simulink model "impmodel"  (R2023a)
settings: Solver=FixedStepDiscrete  StartTime=0.0  StopTime=8  RelTol=1e-3  EnableMultiTasking=on
values from neighbouring files (symbols this model uses):
  availableSpeedModes = 3    [params_f2838.mat]
  inverter_DRV8300 =     [params_f2838.mat]
  PI_params =     [params_f2838.mat]
  pmsm_ECI6360 =     [params_f2838.mat]
  PU_System =     [params_f2838.mat]
  target_f2838 =     [params_f2838.mat]
  Ts = 5e-05    [params_f2838.mat]
  Ts_motor = 2.5e-05    [params_f2838.mat]
  Ts_simulink = 2.5e-05    [params_f2838.mat]
  Ts_speed = 0.0005    [params_f2838.mat]
undefined symbols (not defined in the file or in its folder): Down, GPTRIP1SEL, TZ1, Up
libraries: simulink x35, c2802xlib x11, idelinklib_common x8, procinterlib x8, mcbcontrolslib x8, c280xlib x7, mcbpositiondecoderlib x7, slpidlib x5, svdschedulerlib x4, c2838xlib x2, autolibpmsminterior x1, mcbplantlib x1
(part 3 of 4)

== system impmodel/Torque Controller/Output/CodeGeneration ==
  In1 : Inport
  Demux : Demux  Outputs=6
  Gain : Gain  Gain=target_f2838.PWM_Counter_Period  OutDataTypeStr=fixdt(1,32,17)
  ePWM1 : c2802xlib/ePWM  PwmType=C2000_Type4_F2838x  useModule=ePWM6  ePWMxLINKTBPRD=Not Linked  periodUnits=Clock cycles  timerSource=Specify via dialog  timerPeriod_clk=target_f2838.PWM_Counter_Period  timerPeriod_sec=0.0001  tbshadow=Counter equals to zero  countingMode=Up-Down  phaseActiveEnable=Disable  phaseDirection=Count down after sync  phaseActive=0  synchronizationEnable=off  dcaevt1Sync=off  dcbevt1Sync=off  synchronizationOption=Disable  dcbevt1SyncOut=off  dcaevt1SyncOut=off  cmpdSyncOut=off  cmpcSyncOut=off  cmpbSyncOut=off  zeroSyncOut=on  swfSyncOut=off  perSynchronizationOption=Counter equals to period (CTR=PRD)  clockPrescale=1  HSclockPrescale=1  enswap=off  ePWMxAStatus=on  ePWMxAactionLogic1=Do nothing  ePWMxAactionLogic2=Do nothing  ePWMxAactionLogic3=Clear  ePWMxAactionLogic4=Set  ePWMxAactionLogic5=Do nothing  ePWMxAactionLogic6=Do nothing  ePWMxACSFenable=off  ePWMxACSFvalue=Forcing disable  ePWMxASFreload=Zero  ePWMxBStatus=on  ePWMxBactionLogic1=Do nothing  ePWMxBactionLogic2=Do nothing  ePWMxBactionLogic3=Do nothing  ePWMxBactionLogic4=Do nothing  ePWMxBactionLogic5=Clear  ePWMxBactionLogic6=Set  ePWMxBCSFenable=off  ePWMxBCSFvalue=Forcing disable  ePWMxBSFreload=Zero  ePWNxBOutWay=off  ePWMxLINKCMPA=Not Linked  CMPAUnits=Clock cycles  CMPASource=Input port  CMPAValue_per=50  CMPAValue_clk=floor(target_f2838.PWM_Counter_Period/2)  enCMPAshadow=Counter equals to zero (CTR=Zero)  ePWMxLINKCMPB=Not Linked  CMPBUnits=Clock cycles  CMPBSource=Input port  CMPBValue_per=50  CMPBValue_clk=floor(target_f2838.PWM_Counter_Period/2)  enCMPBshadow=Counter equals to zero (CTR=Zero)  ePWMxLINKCMPC=Not Linked  CMPCUnits=Clock cycles  CMPCSource=Specify via dialog  CMPCValue_per=50  CMPCValue_clk=32000  enCMPCshadow=Counter equals to zero (CTR=Zero)  ePWMxLINKCMPD=Not Linked  CMPDUnits=Clock cycles  CMPDSource=Specify via dialog  CMPDValue_per=50  CMPDValue_clk=32000  enCMPDshadow=Counter equals to zero (CTR=Zero)  enableDBePWMxA=off  enableDBePWMxB=off  enhalfcycle=off  DBpolarity=Active high complementary (AHC)  DBedgeDelay=Positive  DBSource_ePWMxA=ePWMxA  DBSource_ePWMxB=ePWMxA  DBPeriodUnits=Clock cycles  DBperiodSource=Specify via dialog  REDperiod=15  FEDperiod=15  REDperiod_sec=0  FEDperiod_sec=0  LoadModeDBRED=Immediate without using shadow  LoadModeDBFED=Immediate without using shadow  adcstartModuleA=on  adcrequestEventA=First event  adcstartEventA=Digital Compare Module A Event 1 start of conversion (DCAEVT1.soc)  adcstartEventA_type2=Counter equals to period (CTR=PRD)  adcstartModuleB=off  adcrequestEventB=First event  adcstartEventB=Counter equals to zero (CTR=Zero)  adcstartEventB_type2=Counter equals to zero (CTR=Zero)  intEn=off  intPrd=First event  intSel=Counter equals to zero (CTR=Zero)  intSel_type2=Counter equals to zero (CTR=Zero)  hrpe=off  enHRPWM=off  HRPWM_LoadMode=Counter equals to period (CTR=PRD)  HRPWM_CTLMode=Duty or Period control mode  HRPWM_EDGMode=Both edge  hrpeb=off  enHRPWMB=off  HRPWM_LoadModeB=Counter equals to zero (CTR=ZERO)  HRPWM_CTLModeB=Duty or Period control mode  HRPWM_EDGModeB=Both edge  enHRDBRED=off  enHRDBFED=off  enSFO=on  enautoconv=on  chopperEnable=off  chopperFrequency=1  chopperFirstwidth=1  chopperDuty=12.5%  tripZonesource=Specify via dialog  tzselOSHT1=off  tzselOSHT2=off  tzselOSHT3=off  tzselOSHDCAEV1=off  tzselOSHDCBEV1=off  tzselCBC1=off  tzselCBC2=off  tzselCBC3=off  tzselCBCDCAEV2=off  tzselCBCDCBEV2=off  tzselOSHT4=off  tzselOSHT5=off  tzselOSHT6=off  tzselCBC4=off  tzselCBC5=off  tzselCBC6=off  enTzOstIntr=off  enTzCbcIntr=off  enTzDCAEVT1Intr=off  enTzDCAEVT2Intr=off  enTzDCBEVT1Intr=off  enTzDCBEVT2Intr=off  ePWMxAforced=No action  ePWMxBforced=No action  DCAEVT1forced=No action  DCBEVT1forced=No action  DCAEVT2forced=No action  DCBEVT2forced=No action  dcah=Trip Zone 1 input (TZ1)  dcal=Trip Zone 2 input (TZ2)  dcbh=Trip Zone 1 input (TZ1)  dcbl=Trip Zone 2 input (TZ2)  dcah_type2=GPTRIP1SEL/(TZ1)  dcal_type2=GPTRIP1SEL/(TZ1)  dcbh_type2=GPTRIP1SEL/(TZ1)  dcbl_type2=GPTRIP1SEL/(TZ1)  gendcaevt1=Event disabled  gendcaevt2=Event disabled  gendcbevt1=Event disabled  gendcbevt2=Event disabled  dcaevt1src=DCAEVT1 with sync  dcaevt2src=DCAEVT2 with sync  dcbevt1src=DCBEVT1 with sync  dcbevt2src=DCBEVT2 with sync  pulsesel=Counter equals to zero (CTR=Zero)  blankinv=off  blankoffset=0  blankwidth=0  evsrcsel=Filtered version of DCAEVT1 (DCAEVT1FILT)  encape=off
      settings: LibrarySourceBlock=c2838xlib/ePWM
  ePWM2 : c2802xlib/ePWM  PwmType=C2000_Type4_F2838x  useModule=ePWM7  ePWMxLINKTBPRD=Not Linked  periodUnits=Clock cycles  timerSource=Specify via dialog  timerPeriod_clk=target_f2838.PWM_Counter_Period  timerPeriod_sec=0.0001  tbshadow=Counter equals to zero  countingMode=Up-Down  phaseActiveEnable=Set counter to phase value specified via dialog  phaseDirection=Count up after sync  phaseActive=0  synchronizationEnable=off  dcaevt1Sync=off  dcbevt1Sync=off  synchronizationOption=Disable  dcbevt1SyncOut=off  dcaevt1SyncOut=off  cmpdSyncOut=off  cmpcSyncOut=off  cmpbSyncOut=off  zeroSyncOut=off  swfSyncOut=on  perSynchronizationOption=Counter equals to period (CTR=PRD)  clockPrescale=1  HSclockPrescale=1  enswap=off  ePWMxAStatus=on  ePWMxAactionLogic1=Do nothing  ePWMxAactionLogic2=Do nothing  ePWMxAactionLogic3=Clear  ePWMxAactionLogic4=Set  ePWMxAactionLogic5=Do nothing  ePWMxAactionLogic6=Do nothing  ePWMxACSFenable=off  ePWMxACSFvalue=Forcing disable  ePWMxASFreload=Zero  ePWMxBStatus=on  ePWMxBactionLogic1=Do nothing  ePWMxBactionLogic2=Do nothing  ePWMxBactionLogic3=Do nothing  ePWMxBactionLogic4=Do nothing  ePWMxBactionLogic5=Clear  ePWMxBactionLogic6=Set  ePWMxBCSFenable=off  ePWMxBCSFvalue=Forcing disable  ePWMxBSFreload=Zero  ePWNxBOutWay=off  ePWMxLINKCMPA=Not Linked  CMPAUnits=Clock cycles  CMPASource=Input port  CMPAValue_per=50  CMPAValue_clk=floor(target_f2838.PWM_Counter_Period/2)  enCMPAshadow=Counter equals to zero (CTR=Zero)  ePWMxLINKCMPB=Not Linked  CMPBUnits=Clock cycles  CMPBSource=Input port  CMPBValue_per=50  CMPBValue_clk=floor(target_f2838.PWM_Counter_Period/2)  enCMPBshadow=Counter equals to zero (CTR=Zero)  ePWMxLINKCMPC=Not Linked  CMPCUnits=Clock cycles  CMPCSource=Specify via dialog  CMPCValue_per=50  CMPCValue_clk=32000  enCMPCshadow=Counter equals to zero (CTR=Zero)  ePWMxLINKCMPD=Not Linked  CMPDUnits=Clock cycles  CMPDSource=Specify via dialog  CMPDValue_per=50  CMPDValue_clk=32000  enCMPDshadow=Counter equals to zero (CTR=Zero)  enableDBePWMxA=off  enableDBePWMxB=off  enhalfcycle=off  DBpolarity=Active high complementary (AHC)  DBedgeDelay=Positive  DBSource_ePWMxA=ePWMxA  DBSource_ePWMxB=ePWMxA  DBPeriodUnits=Clock cycles  DBperiodSource=Specify via dialog  REDperiod=15  FEDperiod=15  REDperiod_sec=0  FEDperiod_sec=0  LoadModeDBRED=Immediate without using shadow  LoadModeDBFED=Immediate without using shadow  adcstartModuleA=off  adcrequestEventA=First event  adcstartEventA=Digital Compare Module A Event 1 start of conversion (DCAEVT1.soc)  adcstartEventA_type2=Counter equals to zero (CTR=Zero)  adcstartModuleB=off  adcrequestEventB=First event  adcstartEventB=Counter equals to zero (CTR=Zero)  adcstartEventB_type2=Counter equals to zero (CTR=Zero)  intEn=off  intPrd=First event  intSel=Counter equals to zero (CTR=Zero)  intSel_type2=Counter equals to zero (CTR=Zero)  hrpe=off  enHRPWM=off  HRPWM_LoadMode=Counter equals to period (CTR=PRD)  HRPWM_CTLMode=Duty or Period control mode  HRPWM_EDGMode=Both edge  hrpeb=off  enHRPWMB=off  HRPWM_LoadModeB=Counter equals to zero (CTR=ZERO)  HRPWM_CTLModeB=Duty or Period control mode  HRPWM_EDGModeB=Both edge  enHRDBRED=off  enHRDBFED=off  enSFO=on  enautoconv=on  chopperEnable=off  chopperFrequency=1  chopperFirstwidth=1  chopperDuty=12.5%  tripZonesource=Specify via dialog  tzselOSHT1=off  tzselOSHT2=off  tzselOSHT3=off  tzselOSHDCAEV1=off  tzselOSHDCBEV1=off  tzselCBC1=off  tzselCBC2=off  tzselCBC3=off  tzselCBCDCAEV2=off  tzselCBCDCBEV2=off  tzselOSHT4=off  tzselOSHT5=off  tzselOSHT6=off  tzselCBC4=off  tzselCBC5=off  tzselCBC6=off  enTzOstIntr=off  enTzCbcIntr=off  enTzDCAEVT1Intr=off  enTzDCAEVT2Intr=off  enTzDCBEVT1Intr=off  enTzDCBEVT2Intr=off  ePWMxAforced=No action  ePWMxBforced=No action  DCAEVT1forced=No action  DCBEVT1forced=No action  DCAEVT2forced=No action  DCBEVT2forced=No action  dcah=Trip Zone 1 input (TZ1)  dcal=Trip Zone 2 input (TZ2)  dcbh=Trip Zone 1 input (TZ1)  dcbl=Trip Zone 2 input (TZ2)  dcah_type2=GPTRIP1SEL/(TZ1)  dcal_type2=GPTRIP1SEL/(TZ1)  dcbh_type2=GPTRIP1SEL/(TZ1)  dcbl_type2=GPTRIP1SEL/(TZ1)  gendcaevt1=Event disabled  gendcaevt2=Event disabled  gendcbevt1=Event disabled  gendcbevt2=Event disabled  dcaevt1src=DCAEVT1 with sync  dcaevt2src=DCAEVT2 with sync  dcbevt1src=DCBEVT1 with sync  dcbevt2src=DCBEVT2 with sync  pulsesel=Counter equals to zero (CTR=Zero)  blankinv=off  blankoffset=0  blankwidth=0  evsrcsel=Filtered version of DCAEVT1 (DCAEVT1FILT)  encape=off
      settings: LibrarySourceBlock=c2838xlib/ePWM
  ePWM3 : c2802xlib/ePWM  PwmType=C2000_Type4_F2838x  useModule=ePWM8  ePWMxLINKTBPRD=Not Linked  periodUnits=Clock cycles  timerSource=Specify via dialog  timerPeriod_clk=target_f2838.PWM_Counter_Period  timerPeriod_sec=0.0001  tbshadow=Counter equals to zero  countingMode=Up-Down  phaseActiveEnable=Set counter to phase value specified via dialog  phaseDirection=Count up after sync  phaseActive=0  synchronizationEnable=off  dcaevt1Sync=off  dcbevt1Sync=off  synchronizationOption=Disable  dcbevt1SyncOut=off  dcaevt1SyncOut=off  cmpdSyncOut=off  cmpcSyncOut=off  cmpbSyncOut=off  zeroSyncOut=off  swfSyncOut=on  perSynchronizationOption=Counter equals to period (CTR=PRD)  clockPrescale=1  HSclockPrescale=1  enswap=off  ePWMxAStatus=on  ePWMxAactionLogic1=Do nothing  ePWMxAactionLogic2=Do nothing  ePWMxAactionLogic3=Clear  ePWMxAactionLogic4=Set  ePWMxAactionLogic5=Do nothing  ePWMxAactionLogic6=Do nothing  ePWMxACSFenable=off  ePWMxACSFvalue=Forcing disable  ePWMxASFreload=Zero  ePWMxBStatus=on  ePWMxBactionLogic1=Do nothing  ePWMxBactionLogic2=Do nothing  ePWMxBactionLogic3=Do nothing  ePWMxBactionLogic4=Do nothing  ePWMxBactionLogic5=Clear  ePWMxBactionLogic6=Set  ePWMxBCSFenable=off  ePWMxBCSFvalue=Forcing disable  ePWMxBSFreload=Zero  ePWNxBOutWay=off  ePWMxLINKCMPA=Not Linked  CMPAUnits=Clock cycles  CMPASource=Input port  CMPAValue_per=50  CMPAValue_clk=floor(target_f2838.PWM_Counter_Period/2)  enCMPAshadow=Counter equals to zero (CTR=Zero)  ePWMxLINKCMPB=Not Linked  CMPBUnits=Clock cycles  CMPBSource=Input port  CMPBValue_per=50  CMPBValue_clk=floor(target_f2838.PWM_Counter_Period/2)  enCMPBshadow=Counter equals to zero (CTR=Zero)  ePWMxLINKCMPC=Not Linked  CMPCUnits=Clock cycles  CMPCSource=Specify via dialog  CMPCValue_per=50  CMPCValue_clk=32000  enCMPCshadow=Counter equals to zero (CTR=Zero)  ePWMxLINKCMPD=Not Linked  CMPDUnits=Clock cycles  CMPDSource=Specify via dialog  CMPDValue_per=50  CMPDValue_clk=32000  enCMPDshadow=Counter equals to zero (CTR=Zero)  enableDBePWMxA=off  enableDBePWMxB=off  enhalfcycle=off  DBpolarity=Active high complementary (AHC)  DBedgeDelay=Positive  DBSource_ePWMxA=ePWMxA  DBSource_ePWMxB=ePWMxA  DBPeriodUnits=Clock cycles  DBperiodSource=Specify via dialog  REDperiod=15  FEDperiod=15  REDperiod_sec=0  FEDperiod_sec=0  LoadModeDBRED=Immediate without using shadow  LoadModeDBFED=Immediate without using shadow  adcstartModuleA=off  adcrequestEventA=First event  adcstartEventA=Digital Compare Module A Event 1 start of conversion (DCAEVT1.soc)  adcstartEventA_type2=Counter equals to zero (CTR=Zero)  adcstartModuleB=off  adcrequestEventB=First event  adcstartEventB=Counter equals to zero (CTR=Zero)  adcstartEventB_type2=Counter equals to zero (CTR=Zero)  intEn=off  intPrd=First event  intSel=Counter equals to zero (CTR=Zero)  intSel_type2=Counter equals to zero (CTR=Zero)  hrpe=off  enHRPWM=off  HRPWM_LoadMode=Counter equals to period (CTR=PRD)  HRPWM_CTLMode=Duty or Period control mode  HRPWM_EDGMode=Both edge  hrpeb=off  enHRPWMB=off  HRPWM_LoadModeB=Counter equals to zero (CTR=ZERO)  HRPWM_CTLModeB=Duty or Period control mode  HRPWM_EDGModeB=Both edge  enHRDBRED=off  enHRDBFED=off  enSFO=on  enautoconv=on  chopperEnable=off  chopperFrequency=1  chopperFirstwidth=1  chopperDuty=12.5%  tripZonesource=Specify via dialog  tzselOSHT1=off  tzselOSHT2=off  tzselOSHT3=off  tzselOSHDCAEV1=off  tzselOSHDCBEV1=off  tzselCBC1=off  tzselCBC2=off  tzselCBC3=off  tzselCBCDCAEV2=off  tzselCBCDCBEV2=off  tzselOSHT4=off  tzselOSHT5=off  tzselOSHT6=off  tzselCBC4=off  tzselCBC5=off  tzselCBC6=off  enTzOstIntr=off  enTzCbcIntr=off  enTzDCAEVT1Intr=off  enTzDCAEVT2Intr=off  enTzDCBEVT1Intr=off  enTzDCBEVT2Intr=off  ePWMxAforced=No action  ePWMxBforced=No action  DCAEVT1forced=No action  DCBEVT1forced=No action  DCAEVT2forced=No action  DCBEVT2forced=No action  dcah=Trip Zone 1 input (TZ1)  dcal=Trip Zone 2 input (TZ2)  dcbh=Trip Zone 1 input (TZ1)  dcbl=Trip Zone 2 input (TZ2)  dcah_type2=GPTRIP1SEL/(TZ1)  dcal_type2=GPTRIP1SEL/(TZ1)  dcbh_type2=GPTRIP1SEL/(TZ1)  dcbl_type2=GPTRIP1SEL/(TZ1)  gendcaevt1=Event disabled  gendcaevt2=Event disabled  gendcbevt1=Event disabled  gendcbevt2=Event disabled  dcaevt1src=DCAEVT1 with sync  dcaevt2src=DCAEVT2 with sync  dcbevt1src=DCBEVT1 with sync  dcbevt2src=DCBEVT2 with sync  pulsesel=Counter equals to zero (CTR=Zero)  blankinv=off  blankoffset=0  blankwidth=0  evsrcsel=Filtered version of DCAEVT1 (DCAEVT1FILT)  encape=off
      settings: LibrarySourceBlock=c2838xlib/ePWM
  wires:
  In1/1 -> Gain/1
  Demux/1 -> ePWM1/1
  Demux/6 -> ePWM3/2
  Demux/2 -> ePWM1/2
  Demux/5 -> ePWM3/1
  Demux/4 -> ePWM2/2
  Demux/3 -> ePWM2/1
  Gain/1 -> Demux/1

== system impmodel/Torque Controller/Output/Simulation ==
  Input : Inport
  Demux : Demux  Outputs=6
  Mux : Mux  Inputs=3
  Terminator : Terminator
  Terminator1 : Terminator
  Terminator2 : Terminator
  Output : Outport
  wires:
  Demux/5 -> Mux/3
  Demux/4 -> Terminator1/1
  Demux/1 -> Mux/1
  Demux/6 -> Terminator/1
  Demux/2 -> Terminator2/1
  Demux/3 -> Mux/2
  Input/1 -> Demux/1
  Mux/1 -> Output/1

== system impmodel/Torque Controller/Scaling DutyCycles/CodeGen ==
  In1 : Inport
  Constant : Constant  Value=0.5  OutDataTypeStr=fixdt(1,32,17)  SampleTime=-1
  Gain : Gain  Gain=-0.5  RndMeth=Simplest  OutDataTypeStr=Inherit: Same as input
  Sum : Sum  Inputs=|++
  Out1 : Outport
  wires:
  In1/1 -> Gain/1
  Sum/1 -> Out1/1
  Constant/1 -> Sum/2
  Gain/1 -> Sum/1

== system impmodel/Torque Controller/Scaling DutyCycles/Sim ==
  In1 : Inport
  Constant : Constant  Value=0.5  OutDataTypeStr=fixdt(1,32,17)  SampleTime=-1
  Gain : Gain  Gain=-0.5  RndMeth=Simplest  OutDataTypeStr=Inherit: Same as input
  Sum : Sum  Inputs=|++
  Out1 : Outport
  wires:
  In1/1 -> Gain/1
  Sum/1 -> Out1/1
  Constant/1 -> Sum/2
  Gain/1 -> Sum/1

== system impmodel/Torque Controller/TCP_Position/Data_Type_Fixed_Point ==
  In1 : Inport
  Data Type Conversion : DataTypeConversion  OutDataTypeStr=fixdt(1,32,17)  RndMeth=Simplest  SaturateOnIntegerOverflow=off
  Data Type Conversion3 : DataTypeConversion  OutDataTypeStr=uint32  ConvertRealWorld=Stored Integer (SI)  RndMeth=Simplest  SaturateOnIntegerOverflow=off
  Data_Log : Outport
  wires:
  In1/1 -> Data Type Conversion/1
  Data Type Conversion3/1 -> Data_Log/1
  Data Type Conversion/1 -> Data Type Conversion3/1

== system impmodel/Torque Controller/TCP_Speed/Data_Type_Fixed_Point ==
  In1 : Inport
  Data Type Conversion : DataTypeConversion  OutDataTypeStr=fixdt(1,32,17)  RndMeth=Simplest  SaturateOnIntegerOverflow=off
  Data Type Conversion3 : DataTypeConversion  OutDataTypeStr=uint32  ConvertRealWorld=Stored Integer (SI)  RndMeth=Simplest  SaturateOnIntegerOverflow=off
  Data_Log : Outport
  wires:
  In1/1 -> Data Type Conversion/1
  Data Type Conversion3/1 -> Data_Log/1
  Data Type Conversion/1 -> Data Type Conversion3/1

== system impmodel/ADC Offset Function/Calculate ADC Offset /For Iterator Subsystem/If Action Subsystem ==
  In1 : Inport
  In2 : Inport  Port=2
  Action Port : ActionPort  ActionPortLabel=if(u1 > 8)
  Memory : Memory  InheritSampleTime=on
  Memory1 : Memory  InheritSampleTime=on
  Sum : Sum
  Sum1 : Sum
  Out1 : Outport
  Out2 : Outport  Port=2
  wires:
  In1/1 -> Sum/1
  Sum/1 -> Out1/1, Memory/1
  In2/1 -> Sum1/1
  Memory/1 -> Sum/2
  Sum1/1 -> Out2/1, Memory1/1
  Memory1/1 -> Sum1/2

== system impmodel/Input Controller/SpeedCommand_CodeGen/Check for SpeedRef/If Action Subsystem ==
  Action Port : ActionPort  ActionPortLabel=if(u1 > 4000)
  Constant : Constant  Value=4095  OutDataTypeStr=uint16  SampleTime=-1
  Out1 : Outport
  wires:
  Constant/1 -> Out1/1

== system impmodel/Input Controller/SpeedCommand_CodeGen/Check for SpeedRef/If Action Subsystem1 ==
  In1 : Inport
  Action Port : ActionPort  ActionPortLabel=else
  Out1 : Outport
  wires:
  In1/1 -> Out1/1

== system impmodel/Input Controller/Subsystem/TCP_temp/Data_Type_Fixed_Point ==
  In1 : Inport
  Data Type Conversion : DataTypeConversion  OutDataTypeStr=fixdt(1,32,17)  RndMeth=Simplest  SaturateOnIntegerOverflow=off
  Data Type Conversion3 : DataTypeConversion  OutDataTypeStr=uint32  ConvertRealWorld=Stored Integer (SI)  RndMeth=Simplest  SaturateOnIntegerOverflow=off
  Data_Log : Outport
  wires:
  In1/1 -> Data Type Conversion/1
  Data Type Conversion3/1 -> Data_Log/1
  Data Type Conversion/1 -> Data Type Conversion3/1

== system impmodel/Speed Control/Speed calculator/Subsystem/If Action Subsystem ==
  Action Port : ActionPort
  Constant : Constant  OutDataTypeStr=fixdt(1,32,17)  SampleTime=-1
  Out1 : Outport
  wires:
  Constant/1 -> Out1/1

== system impmodel/Speed Control/Speed calculator/Subsystem/If Action Subsystem1 ==
  In1 : Inport
  Action Port : ActionPort
  Data Type Conversion : DataTypeConversion  OutDataTypeStr=fixdt(1,32,17)  SaturateOnIntegerOverflow=off  RndMeth=Floor
  Out1 : Outport
  wires:
  In1/1 -> Data Type Conversion/1
  Data Type Conversion/1 -> Out1/1

== system impmodel/Torque Controller/FOC/Current_Controllers/PI_Controller_Id ==
  Id_in : Inport
  Data Store Read1 : DataStoreRead  Commented=on  DataStoreName=Enable  IndexOptions=Index vector (dialog)  Indices=1  OutputSizes=1
  Discrete PI Controller with anti-windup & reset : slpidlib/PID Controller  Commented=on  Controller=PI  Form=Parallel  TimeDomain=Discrete-time  UseExternalTs=off  SampleTime=-1  IntegratorMethod=Forward Euler  FilterMethod=Forward Euler  ControllerParametersSource=external  P=1  I=1  UseKiTs=on  D=0  N=100  UseFilter=on  TunerSelectOption=Transfer Function Based (PID Tuner App)  InitialConditionSource=external  InitialConditionForIntegrator=0  InitialConditionForFilter=0  DifferentiatorICPrevScaledInput=0  ExternalReset=level  TrackingMode=off  Kt=1  LimitOutput=on  SatLimitsSource=internal  UpperSaturationLimit=1  LowerSaturationLimit=-1  LinearizeAsGain=on  AntiWindupMode=clamping  Kb=1  LimitIntegrator=off  UpperIntegratorSaturationLimit=inf  LowerIntegratorSaturationLimit=-inf  RndMeth=Simplest  PGainOutDataTypeStr=single  PProdOutDataTypeStr=single  POutMin=[]  POutMax=[]  IGainOutDataTypeStr=single  IProdOutDataTypeStr=single  IOutMin=[]  IOutMax=[]  DOutMin=[]  DOutMax=[]  NOutMin=[]  NOutMax=[]  SumOutDataTypeStr=single  SumOutMin=[]  SumOutMax=[]  SaturationOutDataTypeStr=single  SaturationOutMin=[]  SaturationOutMax=[]  PParamMin=[]  PParamMax=[]  IParamMin=[]  IParamMax=[]  DParamMin=[]  DParamMax=[]  NParamMin=[]  NParamMax=[]  KbParamMin=[]  KbParamMax=[]  KtParamMin=[]  KtParamMax=[]  KbOutMin=[]  KbOutMax=[]  KtOutMin=[]  KtOutMax=[]  IntegratorOutMin=[]  IntegratorOutMax=[]  FilterOutMin=[]  FilterOutMax=[]  SumI1OutMin=[]  SumI1OutMax=[]  SumI2OutMin=[]  SumI2OutMax=[]  SumI3OutMin=[]  SumI3OutMax=[]  SumI4OutMin=[]  SumI4OutMax=[]  SumDOutMin=[]  SumDOutMax=[]  DifferentiatorOutMin=[]  DifferentiatorOutMax=[]  FilterDiffOutCoefMin=[]  FilterDiffOutCoefMax=[]  ReciprocalOutMin=[]  ReciprocalOutMax=[]  SumDenOutMin=[]  SumDenOutMax=[]  SumNumOutMin=[]  SumNumOutMax=[]  DivideOutMin=[]  DivideOutMax=[]  UdiffTsProdOutMin=[]  UdiffTsProdOutMax=[]  NTsProdOutMin=[]  NTsProdOutMax=[]  UintegralTsProdOutMin=[]  UintegralTsProdOutMax=[]  UngainTsProdOutMin=[]  UngainTsProdOutMax=[]  ClampingZeroOutDataTypeStr=Inherit: Inherit via back propagation  ClampingZeroOutMin=[]  ClampingZeroOutMax=[]  FilterDenConstantOutDataTypeStr=Inherit: Inherit via back propagation  FilterDenConstantOutMin=[]  FilterDenConstantOutMax=[]  PCopyOutDataTypeStr=Inherit: Inherit via back propagation  PCopyOutMin=[]  PCopyOutMax=[]  NCopyOutDataTypeStr=Inherit: Inherit via back propagation  NCopyOutMin=[]  NCopyOutMax=[]  IntegratorContinuousStateAttributes=''  IntegratorStateMustResolveToSignalObject=off  IntegratorRTWStateStorageClass=Auto  FilterContinuousStateAttributes=''  FilterStateMustResolveToSignalObject=off  FilterRTWStateStorageClass=Auto  ParallelPVariant=ExternalParameters  IdealPVariant=Disabled  IVariant=ExternalParameters  DVariant=Disabled  IntegratorVariant=Discrete  SatVariant=Enabled  AWVariant=DiscClampingParallel  PCopyVariant=Disabled  TRVariant=Disabled  FdbkBlocksVariant=Forward  IdealPFdbkVariant=Disabled  SatFdbkVariant=Disabled  DerivativeFilterVariant=Disabled  NVariant=Disabled  NCopyVariant=Disabled_SignalSpec  FilterICVariant=Disabled  IntegratorICVariant=ExternalICs  ExternalResetVariant=ExternalReset  TRSumVariant=Passthrough  SumFdbkVariant=Disabled  SumVariant=Sum_PI  TsampFilterVariant=InternalTs  TsampNgainVariant=Passthrough  TsampIntegralVariant=Disabled_SignalSpec  ExternalSaturationOutDataTypeStr=Inherit: Same as second input
      settings: LibrarySourceBlock=mcbcontrolslib/PI Controller
  Ki : Constant  Commented=on  Value=PI_params.Ki_id*Ts  OutDataTypeStr=single  SampleTime=-1
  Ki1 : Constant  Commented=on  Value=0  OutDataTypeStr=single  SampleTime=-1
  Kp : Constant  Commented=on  Value=PI_params.Kp_id  OutDataTypeStr=single  SampleTime=-1
  Logical Operator : Logic  Commented=on  Operator=NOT  IconShape=distinctive  AllPortsSameDT=off  OutDataTypeStr=boolean
  PID Controller : slpidlib/PID Controller  Controller=PI  Form=Parallel  TimeDomain=Discrete-time  UseExternalTs=off  SampleTime=-1  IntegratorMethod=Forward Euler  FilterMethod=Forward Euler  ControllerParametersSource=internal  P=PI_params.Kp_id-0.0002  I=PI_params.Ki_d_texas*Ts  UseKiTs=on  D=0  N=100  UseFilter=on  TunerSelectOption=Transfer Function Based (PID Tuner App)  InitialConditionSource=internal  InitialConditionForIntegrator=0  InitialConditionForFilter=0  DifferentiatorICPrevScaledInput=0  ExternalReset=none  TrackingMode=off  Kt=1  LimitOutput=on  SatLimitsSource=internal  UpperSaturationLimit=1  LowerSaturationLimit=0  LinearizeAsGain=off  AntiWindupMode=clamping  Kb=1  LimitIntegrator=off  UpperIntegratorSaturationLimit=inf  LowerIntegratorSaturationLimit=-inf  POutMin=[]  POutMax=[]  IOutMin=[]  IOutMax=[]  DOutMin=[]  DOutMax=[]  NOutMin=[]  NOutMax=[]  SumOutMin=[]  SumOutMax=[]  SaturationOutMin=[]  SaturationOutMax=[]  PParamMin=[]  PParamMax=[]  IParamMin=[]  IParamMax=[]  DParamMin=[]  DParamMax=[]  NParamMin=[]  NParamMax=[]  KbParamMin=[]  KbParamMax=[]  KtParamMin=[]  KtParamMax=[]  KbOutMin=[]  KbOutMax=[]  KtOutMin=[]  KtOutMax=[]  IntegratorOutMin=[]  IntegratorOutMax=[]  FilterOutMin=[]  FilterOutMax=[]  SumI1OutMin=[]  SumI1OutMax=[]  SumI2OutMin=[]  SumI2OutMax=[]  SumI3OutMin=[]  SumI3OutMax=[]  SumI4OutMin=[]  SumI4OutMax=[]  SumDOutMin=[]  SumDOutMax=[]  DifferentiatorOutMin=[]  DifferentiatorOutMax=[]  FilterDiffOutCoefMin=[]  FilterDiffOutCoefMax=[]  ReciprocalOutMin=[]  ReciprocalOutMax=[]  SumDenOutMin=[]  SumDenOutMax=[]  SumNumOutMin=[]  SumNumOutMax=[]  DivideOutMin=[]  DivideOutMax=[]  UdiffTsProdOutMin=[]  UdiffTsProdOutMax=[]  NTsProdOutMin=[]  NTsProdOutMax=[]  UintegralTsProdOutMin=[]  UintegralTsProdOutMax=[]  UngainTsProdOutMin=[]  UngainTsProdOutMax=[]  ClampingZeroOutDataTypeStr=Inherit: Inherit via back propagation  ClampingZeroOutMin=[]  ClampingZeroOutMax=[]  FilterDenConstantOutDataTypeStr=Inherit: Inherit via back propagation  FilterDenConstantOutMin=[]  FilterDenConstantOutMax=[]  PCopyOutDataTypeStr=Inherit: Inherit via back propagation  PCopyOutMin=[]  PCopyOutMax=[]  NCopyOutDataTypeStr=Inherit: Inherit via back propagation  NCopyOutMin=[]  NCopyOutMax=[]  IntegratorContinuousStateAttributes=''  IntegratorStateMustResolveToSignalObject=off  IntegratorRTWStateStorageClass=Auto  FilterContinuousStateAttributes=''  FilterStateMustResolveToSignalObject=off  FilterRTWStateStorageClass=Auto  ParallelPVariant=InternalParameters  IdealPVariant=Disabled  IVariant=InternalParameters  DVariant=Disabled  IntegratorVariant=Discrete  SatVariant=Enabled  AWVariant=DiscClampingParallel  PCopyVariant=Disabled  TRVariant=Disabled  FdbkBlocksVariant=Forward  IdealPFdbkVariant=Disabled  SatFdbkVariant=Disabled  DerivativeFilterVariant=Disabled  NVariant=Disabled  NCopyVariant=Disabled_SignalSpec  FilterICVariant=Disabled  IntegratorICVariant=InternalICs  ExternalResetVariant=Disabled  TRSumVariant=Passthrough  SumFdbkVariant=Disabled  SumVariant=Sum_PI  TsampFilterVariant=InternalTs  TsampNgainVariant=Passthrough  TsampIntegralVariant=Disabled_SignalSpec  ExternalSaturationOutDataTypeStr=Inherit: Same as second input
  V_ref : Outport  VectorParamsAs1DForOutWhenUnconnected=off
  wires:
  Data Store Read1/1 -> Logical Operator/1
  Kp/1 -> Discrete PI Controller with anti-windup & reset/2
  Ki/1 -> Discrete PI Controller with anti-windup & reset/3
  Logical Operator/1 -> Discrete PI Controller with anti-windup & reset/4
  Ki1/1 -> Discrete PI Controller with anti-windup & reset/5
  PID Controller/1 -> V_ref/1
  Id_in/1 -> PID Controller/1

== system impmodel/Torque Controller/FOC/Current_Controllers/PI_Controller_Iq ==
  Iq_in : Inport
  Data Store Read1 : DataStoreRead  Commented=on  DataStoreName=Enable  IndexOptions=Index vector (dialog)  Indices=1  OutputSizes=1
  Discrete PI Controller with anti-windup & reset : slpidlib/PID Controller  Commented=on  Controller=PI  Form=Parallel  TimeDomain=Discrete-time  UseExternalTs=off  SampleTime=-1  IntegratorMethod=Forward Euler  FilterMethod=Forward Euler  ControllerParametersSource=external  P=1  I=1  UseKiTs=on  D=0  N=100  UseFilter=on  TunerSelectOption=Transfer Function Based (PID Tuner App)  InitialConditionSource=external  InitialConditionForIntegrator=0  InitialConditionForFilter=0  DifferentiatorICPrevScaledInput=0  ExternalReset=level  TrackingMode=off  Kt=1  LimitOutput=on  SatLimitsSource=internal  UpperSaturationLimit=1  LowerSaturationLimit=-1  LinearizeAsGain=on  AntiWindupMode=clamping  Kb=1  LimitIntegrator=off  UpperIntegratorSaturationLimit=inf  LowerIntegratorSaturationLimit=-inf  RndMeth=Simplest  POutMin=[]  POutMax=[]  IOutMin=[]  IOutMax=[]  DOutMin=[]  DOutMax=[]  NOutMin=[]  NOutMax=[]  SumOutMin=[]  SumOutMax=[]  SaturationOutDataTypeStr=Inherit: Inherit via back propagation  SaturationOutMin=[]  SaturationOutMax=[]  PParamMin=[]  PParamMax=[]  IParamMin=[]  IParamMax=[]  DParamMin=[]  DParamMax=[]  NParamMin=[]  NParamMax=[]  KbParamMin=[]  KbParamMax=[]  KtParamMin=[]  KtParamMax=[]  KbOutMin=[]  KbOutMax=[]  KtOutMin=[]  KtOutMax=[]  IntegratorOutMin=[]  IntegratorOutMax=[]  FilterOutMin=[]  FilterOutMax=[]  SumI1OutMin=[]  SumI1OutMax=[]  SumI2OutMin=[]  SumI2OutMax=[]  SumI3OutMin=[]  SumI3OutMax=[]  SumI4OutMin=[]  SumI4OutMax=[]  SumDOutMin=[]  SumDOutMax=[]  DifferentiatorOutMin=[]  DifferentiatorOutMax=[]  FilterDiffOutCoefMin=[]  FilterDiffOutCoefMax=[]  ReciprocalOutMin=[]  ReciprocalOutMax=[]  SumDenOutMin=[]  SumDenOutMax=[]  SumNumOutMin=[]  SumNumOutMax=[]  DivideOutMin=[]  DivideOutMax=[]  UdiffTsProdOutMin=[]  UdiffTsProdOutMax=[]  NTsProdOutMin=[]  NTsProdOutMax=[]  UintegralTsProdOutMin=[]  UintegralTsProdOutMax=[]  UngainTsProdOutMin=[]  UngainTsProdOutMax=[]  ClampingZeroOutDataTypeStr=Inherit: Inherit via back propagation  ClampingZeroOutMin=[]  ClampingZeroOutMax=[]  FilterDenConstantOutDataTypeStr=Inherit: Inherit via back propagation  FilterDenConstantOutMin=[]  FilterDenConstantOutMax=[]  PCopyOutDataTypeStr=Inherit: Inherit via back propagation  PCopyOutMin=[]  PCopyOutMax=[]  NCopyOutDataTypeStr=Inherit: Inherit via back propagation  NCopyOutMin=[]  NCopyOutMax=[]  IntegratorContinuousStateAttributes=''  IntegratorStateMustResolveToSignalObject=off  IntegratorRTWStateStorageClass=Auto  FilterContinuousStateAttributes=''  FilterStateMustResolveToSignalObject=off  FilterRTWStateStorageClass=Auto  ParallelPVariant=ExternalParameters  IdealPVariant=Disabled  IVariant=ExternalParameters  DVariant=Disabled  IntegratorVariant=Discrete  SatVariant=Enabled  AWVariant=DiscClampingParallel  PCopyVariant=Disabled  TRVariant=Disabled  FdbkBlocksVariant=Forward  IdealPFdbkVariant=Disabled  SatFdbkVariant=Disabled  DerivativeFilterVariant=Disabled  NVariant=Disabled  NCopyVariant=Disabled_SignalSpec  FilterICVariant=Disabled  IntegratorICVariant=ExternalICs  ExternalResetVariant=ExternalReset  TRSumVariant=Passthrough  SumFdbkVariant=Disabled  SumVariant=Sum_PI  TsampFilterVariant=InternalTs  TsampNgainVariant=Passthrough  TsampIntegralVariant=Disabled_SignalSpec  ExternalSaturationOutDataTypeStr=Inherit: Same as second input
      settings: LibrarySourceBlock=mcbcontrolslib/PI Controller
  Ki : Constant  Commented=on  Value=PI_params.Ki_i*Ts  OutDataTypeStr=single  SampleTime=-1
  Kp : Constant  Commented=on  Value=PI_params.Kp_i  OutDataTypeStr=single  SampleTime=-1
  Kp1 : Constant  Commented=on  Value=0  OutDataTypeStr=single  SampleTime=-1
  Logical Operator : Logic  Commented=on  Operator=NOT  IconShape=distinctive  AllPortsSameDT=off  OutDataTypeStr=boolean
  PID Controller : slpidlib/PID Controller  Controller=PI  Form=Parallel  TimeDomain=Discrete-time  UseExternalTs=off  SampleTime=-1  IntegratorMethod=Forward Euler  FilterMethod=Forward Euler  ControllerParametersSource=internal  P=PI_params.Kp_i-0.0002  I=PI_params.Ki_texas*Ts  UseKiTs=on  D=0  N=100  UseFilter=on  TunerSelectOption=Transfer Function Based (PID Tuner App)  InitialConditionSource=internal  InitialConditionForIntegrator=0  InitialConditionForFilter=0  DifferentiatorICPrevScaledInput=0  ExternalReset=none  TrackingMode=off  Kt=1  LimitOutput=on  SatLimitsSource=internal  UpperSaturationLimit=1  LowerSaturationLimit=0  LinearizeAsGain=off  AntiWindupMode=clamping  Kb=1  LimitIntegrator=off  UpperIntegratorSaturationLimit=inf  LowerIntegratorSaturationLimit=-inf  POutMin=[]  POutMax=[]  IOutMin=[]  IOutMax=[]  DOutMin=[]  DOutMax=[]  NOutMin=[]  NOutMax=[]  SumOutMin=[]  SumOutMax=[]  SaturationOutMin=[]  SaturationOutMax=[]  PParamMin=[]  PParamMax=[]  IParamMin=[]  IParamMax=[]  DParamMin=[]  DParamMax=[]  NParamMin=[]  NParamMax=[]  KbParamMin=[]  KbParamMax=[]  KtParamMin=[]  KtParamMax=[]  KbOutMin=[]  KbOutMax=[]  KtOutMin=[]  KtOutMax=[]  IntegratorOutMin=[]  IntegratorOutMax=[]  FilterOutMin=[]  FilterOutMax=[]  SumI1OutMin=[]  SumI1OutMax=[]  SumI2OutMin=[]  SumI2OutMax=[]  SumI3OutMin=[]  SumI3OutMax=[]  SumI4OutMin=[]  SumI4OutMax=[]  SumDOutMin=[]  SumDOutMax=[]  DifferentiatorOutMin=[]  DifferentiatorOutMax=[]  FilterDiffOutCoefMin=[]  FilterDiffOutCoefMax=[]  ReciprocalOutMin=[]  ReciprocalOutMax=[]  SumDenOutMin=[]  SumDenOutMax=[]  SumNumOutMin=[]  SumNumOutMax=[]  DivideOutMin=[]  DivideOutMax=[]  UdiffTsProdOutMin=[]  UdiffTsProdOutMax=[]  NTsProdOutMin=[]  NTsProdOutMax=[]  UintegralTsProdOutMin=[]  UintegralTsProdOutMax=[]  UngainTsProdOutMin=[]  UngainTsProdOutMax=[]  ClampingZeroOutDataTypeStr=Inherit: Inherit via back propagation  ClampingZeroOutMin=[]  ClampingZeroOutMax=[]  FilterDenConstantOutDataTypeStr=Inherit: Inherit via back propagation  FilterDenConstantOutMin=[]  FilterDenConstantOutMax=[]  PCopyOutDataTypeStr=Inherit: Inherit via back propagation  PCopyOutMin=[]  PCopyOutMax=[]  NCopyOutDataTypeStr=Inherit: Inherit via back propagation  NCopyOutMin=[]  NCopyOutMax=[]  IntegratorContinuousStateAttributes=''  IntegratorStateMustResolveToSignalObject=off  IntegratorRTWStateStorageClass=Auto  FilterContinuousStateAttributes=''  FilterStateMustResolveToSignalObject=off  FilterRTWStateStorageClass=Auto  ParallelPVariant=InternalParameters  IdealPVariant=Disabled  IVariant=InternalParameters  DVariant=Disabled  IntegratorVariant=Discrete  SatVariant=Enabled  AWVariant=DiscClampingParallel  PCopyVariant=Disabled  TRVariant=Disabled  FdbkBlocksVariant=Forward  IdealPFdbkVariant=Disabled  SatFdbkVariant=Disabled  DerivativeFilterVariant=Disabled  NVariant=Disabled  NCopyVariant=Disabled_SignalSpec  FilterICVariant=Disabled  IntegratorICVariant=InternalICs  ExternalResetVariant=Disabled  TRSumVariant=Passthrough  SumFdbkVariant=Disabled  SumVariant=Sum_PI  TsampFilterVariant=InternalTs  TsampNgainVariant=Passthrough  TsampIntegralVariant=Disabled_SignalSpec  ExternalSaturationOutDataTypeStr=Inherit: Same as second input
  V_ref : Outport  VectorParamsAs1DForOutWhenUnconnected=off
  wires:
  Data Store Read1/1 -> Logical Operator/1
  Kp/1 -> Discrete PI Controller with anti-windup & reset/2
  Ki/1 -> Discrete PI Controller with anti-windup & reset/3
  Logical Operator/1 -> Discrete PI Controller with anti-windup & reset/4
  Kp1/1 -> Discrete PI Controller with anti-windup & reset/5
  PID Controller/1 -> V_ref/1
  Iq_in/1 -> PID Controller/1

== system impmodel/Torque Controller/Input Scaling/CodeGeneration/Calculate Position from Hall ==
  Atomic Hall Reading : Subsystem
  Data Store Write : DataStoreWrite  DataStoreName=HallStateChangeFlag  IndexOptions=Index vector (dialog)  Indices=1  OutputSizes=1
  Glitch Filter : simulink/Logic and Bit Operations/Compare To Constant  relop=>=  const=target_f2838.CPU_frequency * 600 / (pmsm_ECI6360.N_base * 10 * 2 * pmsm_ECI6360.p)  OutDataTypeStr=boolean
  Hall Speed and Position : mcbpositiondecoderlib/Hall Speed and Position  blkExecutionType=Speed and position  CounterSize=32 bits  ClkFreq=target_f2838.CPU_frequency  BlkSampleTime=Ts  PolePairs=pmsm_ECI6360.p  MinSpeed=20  HallInterruptConfig=Every 180 Degrees  SpeedUnit=Per unit  PerUnitSpeed=PU_System.N_base  SpeedDataType=fixdt(1,32,17)  hallSequence=ABC  Sequence=[5,4,6,2,3,1]  EnableSecondOrder=1st Order  PositionUnit=Per unit  PositionDataType=fixdt(1,32,17)
      settings: LibrarySourceBlock=mcblib/Sensor Decoders/Hall Speed and Position
  Mechanical to Electrical Position : mcbpositiondecoderlib/Mechanical to Electrical Position  NrPP=1  selectedRange=Per unit  MechOfstInputType=Specify via dialog  mechOffsetIn=0.38  maxAngleIn=1  InputDataType=fixdt(1,32,17)  VariantSelect=floating-point
      settings: LibrarySourceBlock=mcblib/Sensor Decoders/Mechanical to Electrical Position
  Subsystem : Subsystem
  Pos_PU : Outport
  Speed_PU : Outport  Port=2
  wires:
  Atomic Hall Reading/6(HallChange) -> Hall Speed and Position/6
  Hall Speed and Position/3 -> Data Store Write/1
  Atomic Hall Reading/5(SpeedValidity) -> Hall Speed and Position/5
  Atomic Hall Reading/2(Count) -> Hall Speed and Position/2
  Atomic Hall Reading/4(Direction) -> Hall Speed and Position/4
  Atomic Hall Reading/1(HallState) -> Hall Speed and Position/1
  Hall Speed and Position/1 -> Mechanical to Electrical Position/1
  Mechanical to Electrical Position/1 -> Pos_PU/1
  Glitch Filter/1 -> Subsystem/Enable
  Atomic Hall Reading/3(SpeedCount) -> Subsystem/1(Input), Glitch Filter/1
  Subsystem/1(Output) -> Hall Speed and Position/3
  Hall Speed and Position/2 -> Speed_PU/1

== system impmodel/Torque Controller/Input Scaling/CodeGeneration/Convert ADC value to PU ==
  note: Shift Gain mit 2hoch9 und fixdt(1,32,20) einmal versuchen
  Iab_ADC : Inport
  Add : Sum  Inputs=+-
  Data Store Read : DataStoreRead  DataStoreName=IaOffset  IndexOptions=Index vector (dialog)  Indices=1  OutputSizes=1
  Data Store Read1 : DataStoreRead  DataStoreName=IbOffset  IndexOptions=Index vector (dialog)  Indices=1  OutputSizes=1
  Data Type Conversion : DataTypeConversion  OutDataTypeStr=int32  ConvertRealWorld=Stored Integer (SI)  SaturateOnIntegerOverflow=off  RndMeth=Floor
  Data Type Conversion1 : DataTypeConversion  OutDataTypeStr=fixdt(1,32,17)  ConvertRealWorld=Stored Integer (SI)  SaturateOnIntegerOverflow=off  RndMeth=Floor
  Display{,1..3} (4 alike) : Display
  Mux : Mux  Inputs=2
  Shift Arithmetic : ArithShift  BitShiftNumber=-6
  Iab_PU : Outport
  wires:
  Iab_ADC/1 -> Data Type Conversion/1
  Data Type Conversion/1 -> Display3/1, Add/1
  Mux/1 -> Add/2
  Add/1 -> Display2/1, Shift Arithmetic/1
  Shift Arithmetic/1 -> Display1/1, Data Type Conversion1/1
  Data Type Conversion1/1 -> Iab_PU/1, Display/1
  Data Store Read/1 -> Mux/1
  Data Store Read1/1 -> Mux/2

== system impmodel/Torque Controller/Input Scaling/Simulation/Convert Iab to PU ==
  Iab_ADC_Sim : Inport
  Add : Sum  Inputs=+-
  Constant : Constant  Value=[inverter_DRV8300.CtSensAOffset inverter_DRV8300.CtSensBOffset]  SampleTime=-1
  Current Sense Gain : Gain  Commented=on  Gain=PU_System.I_base/1.65  RndMeth=Simplest  OutDataTypeStr=Inherit: Same as input
  Data Type Conversion : DataTypeConversion  OutDataTypeStr=int32  ConvertRealWorld=Stored Integer (SI)  SaturateOnIntegerOverflow=off  RndMeth=Floor
  Data Type Conversion1 : DataTypeConversion  OutDataTypeStr=fixdt(1,32,17)  ConvertRealWorld=Stored Integer (SI)  RndMeth=Simplest  SaturateOnIntegerOverflow=off
  Get_ADC_Volt : Gain  Commented=on  Gain=1.65/(4096/2)  OutDataTypeStr=double  RndMeth=Simplest
  PU_Conversion : Gain  Commented=on  Gain=1/PU_System.I_base  RndMeth=Simplest  OutDataTypeStr=Inherit: Same as input
  Shift Arithmetic : ArithShift  BitShiftNumber=-6
  Iab_PU : Outport
  wires:
  Iab_ADC_Sim/1 -> Data Type Conversion/1
  Data Type Conversion/1 -> Add/1
  Constant/1 -> Add/2
  Data Type Conversion1/1 -> Iab_PU/1
  Shift Arithmetic/1 -> Data Type Conversion1/1
  Add/1 -> Shift Arithmetic/1
  Current Sense Gain/1 -> PU_Conversion/1
  Get_ADC_Volt/1 -> Current Sense Gain/1

== system impmodel/Torque Controller/Input Scaling/Simulation/Convert Pos to PU ==
  Pos_Sim : Inport
  IIR Filter : mcbcontrolslib/IIR Filter  VariantControl=Low Pass Filter  VariantSelect=Low-pass  Filter_constant=0.2  advancedSettings=off  Ts=50e-6  cutOff_freq=795.7747
      settings: LibrarySourceBlock=mcbhdllib/Signal Management/IIR Filter
  Mechanical to Electrical Position : mcbpositiondecoderlib/Mechanical to Electrical Position  NrPP=pmsm_ECI6360.p  selectedRange=Per unit  MechOfstInputType=Specify via dialog  mechOffsetIn=0.38  maxAngleIn=1  InputDataType=fixdt(1,32,17)  VariantSelect=floating-point
      settings: LibrarySourceBlock=mcblib/Sensor Decoders/Mechanical to Electrical Position
  Speed Measurement : mcbpositiondecoderlib/Speed Measurement  PositionUnit=Per unit  PositionScalingDatatype=uint32  SpeedCalculationMode=Time interval for speed calculation  SampleTimeAsync=Ts  MaximumApplicationSpeed=1000  SpeedResolution=5e-6  DelayLength=10  MaximumMeasurableSpeed=59999  MeasurableSpeedResolution=2.794e-05  SpeedUnit=Per unit based on dialog  PerUnitSpeed=PU_System.N_base  SpeedDataType=fixdt(1,32,17)
      settings: LibrarySourceBlock=mcblib/Sensor Decoders/Speed Measurement
  Theta : Outport
  Speed_PU : Outport  Port=2
  wires:
  Pos_Sim/1 -> Mechanical to Electrical Position/1, Speed Measurement/1
  Speed Measurement/1 -> IIR Filter/1
  Mechanical to Electrical Position/1 -> Theta/1
  IIR Filter/1 -> Speed_PU/1

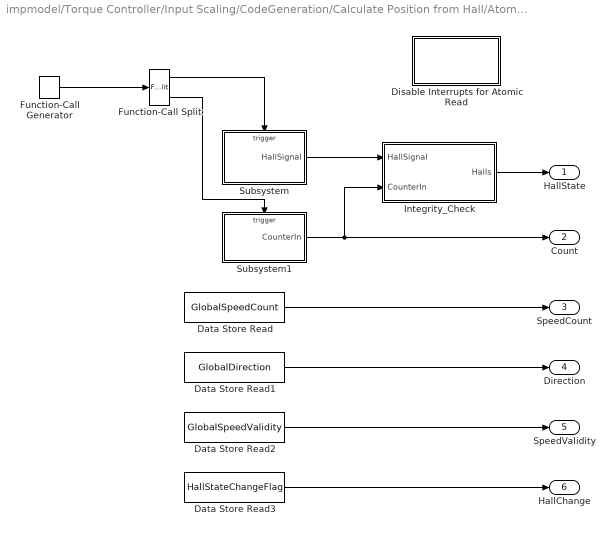
== system impmodel/Torque Controller/Input Scaling/CodeGeneration/Calculate Position from Hall/Atomic Hall Reading ==
  Data Store Read : DataStoreRead  DataStoreName=GlobalSpeedCount  IndexOptions=Index vector (dialog)  Indices=1  OutputSizes=1
  Data Store Read1 : DataStoreRead  DataStoreName=GlobalDirection  IndexOptions=Index vector (dialog)  Indices=1  OutputSizes=1
  Data Store Read2 : DataStoreRead  DataStoreName=GlobalSpeedValidity  IndexOptions=Index vector (dialog)  Indices=1  OutputSizes=1
  Data Store Read3 : DataStoreRead  DataStoreName=HallStateChangeFlag  IndexOptions=Index vector (dialog)  Indices=1  OutputSizes=1
  Disable Interrupts for Atomic Read : Subsystem  mask(System Outputs){ShowInLibBrowser=0}
      mask prompts: ShowInLibBrowser "Simulink:masks:CustCodeMaskParam1_MP"
      settings: CopyFcn=cccopyfcn(gcb)  OpenFcn=ccopenfcn('System Outputs Function')
      mask Help: eval('feval(''rtwprivate'',''rtwhelpview'',''rtw_sys_outputs_block'')');
      mask Display: disp('System\nOutputs');
  Function-Call Generator : simulink/Ports & Subsystems/Function-Call Generator  sample_time=-1  numberOfIterations=1  DisallowWideOutput=off
  Function-Call Split : FunctionCallSplit  IconShape=distinctive  NumOutputPorts=2  OutputPortLayout=default
  Integrity_Check : Subsystem
  Subsystem : Subsystem
  Subsystem1 : Subsystem
  HallState : Outport
  Count : Outport  Port=2
  SpeedCount : Outport  Port=3
  Direction : Outport  Port=4
  SpeedValidity : Outport  Port=5
  HallChange : Outport  Port=6
  wires:
  Function-Call Generator/1 -> Function-Call Split/1
  Data Store Read2/1 -> SpeedValidity/1
  Data Store Read3/1 -> HallChange/1
  Data Store Read1/1 -> Direction/1
  Data Store Read/1 -> SpeedCount/1
  Subsystem/1(HallSignal) -> Integrity_Check/1(HallSignal)
  Integrity_Check/1(Halls) -> HallState/1
  Function-Call Split/2 -> Subsystem1/Trigger
  Function-Call Split/1 -> Subsystem/Trigger
  Subsystem1/1(CounterIn) -> Count/1, Integrity_Check/2(CounterIn)

== system impmodel/Torque Controller/Input Scaling/CodeGeneration/Calculate Position from Hall/Subsystem ==
  Input : Inport
  Enable : EnablePort
  Output : Outport
  wires:
  Input/1 -> Output/1

== system impmodel/Torque Controller/Input Scaling/CodeGeneration/Calculate Position from Hall/Atomic Hall Reading/Disable Interrupts for Atomic Read ==

== system impmodel/Torque Controller/Input Scaling/CodeGeneration/Calculate Position from Hall/Atomic Hall Reading/Integrity_Check ==
  HallSignal : Inport
  CounterIn : Inport  Port=2
  Compare To Constant : simulink/Logic and Bit Operations/Compare To Constant  relop=<=  const=2500  OutDataTypeStr=boolean
  Display1 : Display
  If : If  IfExpression=u1 == 0
  Merge : Merge
  NOT : Logic  AllPortsSameDT=off  OutDataTypeStr=boolean
  No_Integrity_issue : Subsystem  TreatAsAtomicUnit=on
  Refresh_Halls : Subsystem  TreatAsAtomicUnit=on
  Relational Operator : RelationalOperator  Operator===  OutDataTypeStr=boolean  RndMeth=Simplest  InputSameDT=off
  Unit Delay : UnitDelay  SampleTime=-1  HasFrameUpgradeWarning=on
  Halls : Outport
  wires:
  Refresh_Halls/1(Out1) -> Merge/2
  HallSignal/1 -> Display1/1, Relational Operator/1, No_Integrity_issue/1(Counter), Unit Delay/1
  If/2 -> Refresh_Halls/Action
  Merge/1 -> Halls/1
  No_Integrity_issue/1(Out1) -> Merge/1
  If/1 -> No_Integrity_issue/Action
  CounterIn/1 -> Compare To Constant/1
  Compare To Constant/1 -> NOT/2
  Relational Operator/1 -> NOT/1
  NOT/1 -> If/1
  Unit Delay/1 -> Relational Operator/2

== system impmodel/Torque Controller/Input Scaling/CodeGeneration/Calculate Position from Hall/Atomic Hall Reading/Subsystem ==
  function call : TriggerPort  TriggerType=function-call  VariantControl=(inherit)  PortDimensions=1
  Bitwise OR : simulink/Logic and Bit Operations/Bitwise Operator  logicop=OR  UseBitMask=off  NumInputPorts=3  BitMask=bin2dec('11011001')  BitMaskRealWorld=Stored Integer
      settings: LibrarySourceBlock=|
      | simulink/Quick Insert/Logic and Bit
      | Operations/Bitwise OR
  Data Type Conversion : DataTypeConversion  OutDataTypeStr=uint32  ConvertRealWorld=Stored Integer (SI)  SaturateOnIntegerOverflow=off  RndMeth=Floor
  GPIO 24 Hall_A : simulink/Logic and Bit Operations/Bitwise Operator  logicop=AND  UseBitMask=on  BitMask=hex2dec('1000000')  BitMaskRealWorld=Stored Integer
      settings: LibrarySourceBlock=|
      | simulink/Quick Insert/Logic and Bit
      | Operations/Bitwise AND
  GPIO 25 Hall_B : simulink/Logic and Bit Operations/Bitwise Operator  logicop=AND  UseBitMask=on  BitMask=hex2dec('2000000')  BitMaskRealWorld=Stored Integer
      settings: LibrarySourceBlock=|
      | simulink/Quick Insert/Logic and Bit
      | Operations/Bitwise AND
  GPIO 26 Hall_C : simulink/Logic and Bit Operations/Bitwise Operator  logicop=AND  UseBitMask=on  BitMask=hex2dec('4000000')  BitMaskRealWorld=Stored Integer
      settings: LibrarySourceBlock=|
      | simulink/Quick Insert/Logic and Bit
      | Operations/Bitwise AND
  Memory Copy : idelinklib_common/Memory Copy  copyFrom=Specified source code symbol  copyFromAddressSource=Specify via dialog  copyFromAddress=hex2dec('00001000')  copyFromSrcCode=&GpioDataRegs.GPADAT.all  dataTypeFrom=uint32  dataDimensionFrom=1  useOffsetFrom=off  offsetFromSrc=Specify via dialog  offsetFrom=0  strideFrom=1  copyTo=Output port  copyToAddressSource=Specify via dialog  copyToAddress=hex2dec('00002000')  copyToSrcCode=myVariableDst  dataTypeTo=uint32  useOffsetTo=off  offsetToSrc=Specify via dialog  offsetTo=0  strideTo=1  sampleTime=-1  useInitValue=off  initValueSrc=Specify constant value  initValue=1  initValueSrcCode=myInitValueVariable  useAsMask=off  maskOperator=bitwise AND  useTermValue=off  termValue=1  isRealtimeEnabled=off  emitCCBeforeWrite=off  CCBeforeWrite=/* Custom Code Before Write*/  emitCCAfterWrite=off  CCAfterWrite=/* Custom Code After Write*/
  Shift Arithmetic : ArithShift  BitShiftNumber=26
  Shift Arithmetic1 : ArithShift  BitShiftNumber=24
  Shift Arithmetic2 : ArithShift  BitShiftNumber=22
  HallSignal : Outport
  wires:
  Data Type Conversion/1 -> HallSignal/1
  Shift Arithmetic2/1 -> Bitwise OR/3
  Shift Arithmetic1/1 -> Bitwise OR/2
  Memory Copy/1 -> GPIO 24 Hall_A/1, GPIO 26 Hall_C/1, GPIO 25 Hall_B/1
  Shift Arithmetic/1 -> Bitwise OR/1
  Bitwise OR/1 -> Data Type Conversion/1
  GPIO 24 Hall_A/1 -> Shift Arithmetic2/1
  GPIO 25 Hall_B/1 -> Shift Arithmetic1/1
  GPIO 26 Hall_C/1 -> Shift Arithmetic/1
